simulink model "LED_PWM"  (Simulink 7.5)
settings: Solver=FixedStepDiscrete  SolverMode=SingleTasking  StartTime=0.0  StopTime=10.0  FixedStep=0.001  RelTol=1e-3
libraries: dsPICdrivers x8
settings Model: Creator=oded  LastModifiedBy=oded
settings OptimizationCC: OptimizeModelRefInitCode=on  LifeSpan=1
settings HardwareCC: ProdBitPerInt=16  ProdEndianess=LittleEndian  ProdWordSize=16  ProdHWDeviceType=16-bit Generic
settings RTWCC: SystemTargetFile=dspic.tlc  MakeCommand=make_CreateMPLAB  TemplateMakefile=dspic_pic30_gcc.tmf  PostCodeGenCommand=dsPIC_Compile()  Description=Embedded Target for Microchip dsPIC (real-time)  ProcessScript=dspic_make_rtw_hook
settings CodeAppCC: IgnoreCustomStorageClasses=off
settings STFCustomTargetCC: IncludeMdlTerminateFcn=off  CombineOutputUpdateFcns=on  SuppressErrorStatus=on  ERTCustomFileBanners=on  SupportContinuousTime=off  SupportNonInlinedSFcns=off  SystemTargetFile=dspic.tlc
settings ERTTargetCC: MultiwordLength=2048  ParMdlRefBuildCompliant=off  CompOptLevelCompliant=off  IncludeMdlTerminateFcn=off  SuppressErrorStatus=on  ERTFirstTimeCompliant=off  ModelStepFunctionPrototypeControlCompliant=off  CPPClassGenCompliant=off  InlinedParameterPlacement=NonHierarchical  ERTSrcFileBannerTemplate=dsPIC_code_template.cgt  ERTHdrFileBannerTemplate=dsPIC_code_template.cgt  ERTDataSrcFileTemplate=dsPIC_code_template.cgt  ERTDataHdrFileTemplate=dsPIC_code_template.cgt  ERTCustomFileTemplate=dsPIC_main.tlc  ConvertIfToSwitch=off
settings CustomProperty: DataType=string  Value=C:\PROGRA~1\MATLAB\R2010a\bin\win32\gmake

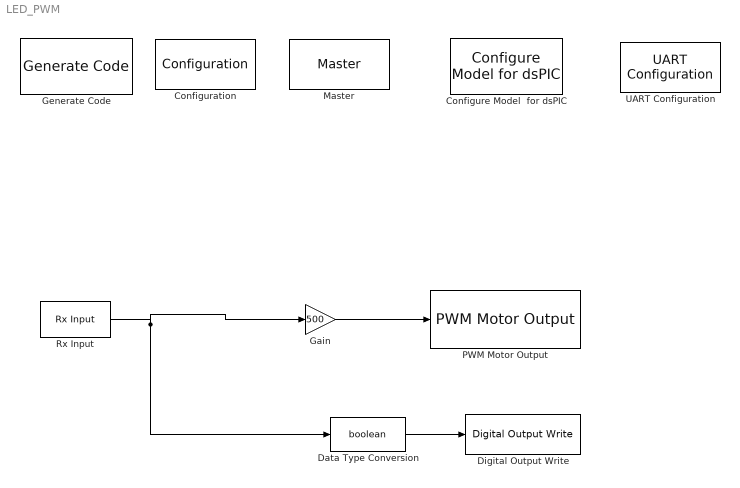
== system LED_PWM ==
  Configuration : dsPICdrivers/Configuration  SystemSampleTime=-1  double64=off
  Configure Model  for dsPIC : dsPICdrivers/Simulink Configuration/Configure Model  for dsPIC
  Data Type Conversion : DataTypeConversion  OutDataTypeMode=boolean  OutDataType=fixdt(1, 16)  OutScaling=2^0  OutDataTypeStr=boolean
  Digital Output Write : dsPICdrivers/Digital I//O/Digital Output Write  Tag=dsPIC_Digital_Output  Priority=5  PORT=B  Pin=[0]  Simultaneous=on  OrderingInOutPopup=None
  Gain : Gain  Gain=500  ParameterDataType=fixdt(1, 16)  ParameterScaling=2^0  OutDataTypeMode=uint16  OutDataType=fixdt(1, 16)  OutScaling=2^0  OutDataTypeStr=uint16
  Generate Code : dsPICdrivers/Simulink Configuration/Generate Code
  Master : dsPICdrivers/Master  Tag=dsPIC_MASTER  Priority=1  TimeStepType=Timer1  picType=30f4011  fcy=5e6  Quartz_33f=5e6  PLLActive_33f=off  fcyDesired_33f=0  tmr1="[1  4999  0]"  tmr1Info="Time Step : 0.001  ;   Error : 0%  PR1=4999"  tmr2345="[0  0  0  0]"  tmr2345cfg=[-1 -1 -1 -1]  IOautoConf=on  typePort="[ 0   0   0   0   0   0   0   0   0   0   0   0   0   0   0   0  10   0   0   0   0   0   0   0   0   0   0   0   0   0   0   0   0   0   0   0   0   0   0   0   0   0   0   0   0   0   0   0   0   0   0   0   0   0   0   0   0   0   0   0   0   0   0   0  11   0   0   0   0   0   0   0   0   0   0   0   0   0   0   0   0   0   0   0   4   5   0   0   0   0   0   0   0   0   0   0   0   0   0   0   0   0   0   0   0   0   0   0   0   0   0   0 ]"  TRIS="[ 65535  65534  65535  65535  65535  65535  65535 ]"  ADPCFG=1  MasterBusyPort=None  MasterOverloadPort=None  FOSC=HS  ClockSwitchMonitor=Both disabled  TempProtection_33f=TEMP_ON  FPBOR=PBOR_OFF  PWRT=PWRT_OFF  MCLR=MCLR_EN  ICD=ICS_PGD1  JTAGEN=JTAGEN_OFF  PowerSave=off  OverrideFcy=off  NewFcy=1e6  PR2345="[65535  65535  65535  65535]"
  PWM Motor Output : dsPICdrivers/Peripheral I//O/PWM Motor Output  Tag=dsPIC_PWM_Motor  Priority=5  PWMref=1  PWM12=1  InputEnableChk=off  InputPeriodeChk=off  Channel=[1 ]  TPeriode=0.02  PrescalerValue=4  PeriodeInteger=25000  MaxName='PWM'  Centered=off  HChannelON=off  Info="Nbr Bits : 15.6096  ||  PWM = 50000  ||  Prescaler = 4"  Delay=0  IntPriority=5  nbrPwmChannelPIC=3  Status=OK  DeadTimePrescaleA=0  DeadTimePrescaleB=0  DeadTimeInfo=Dead Time A = 0  DTPWM1a=Prescaler A  DTPWM1i=Prescaler A  DTPWM2a=Prescaler A  DTPWM2i=Prescaler A  DTPWM3a=Prescaler A  DTPWM3i=Prescaler A  DTPWM4a=Prescaler A  DTPWM4i=Prescaler A  DTCON1=0  DTCON2=0
  Rx Input : dsPICdrivers/Serial PORT/Rx Input  Tag=dsPIC_RX  Priority=5  UART=2  SampleTime=-1  BlockingFctChk=on  OutputDefault=0  IsPresentFlagChk=off  OrderingInOutPopup=None
  UART Configuration : dsPICdrivers/Serial PORT/UART Configuration  Tag=dsPIC_config_UART  Priority=2  UART=2  proposed_BAUD=9600  BAUD=9600  ALT_TX_RX=off  InterruptTxWhen=Do not use interrupt  TXInterruptPri=7  TxBufferSize=32  TXEN=on  InterruptRxWhen=Do not use interrupt  RXInterruptPri=2  RxBufferSize=32  DoNotImplementRxInterrupt=on  DoNotImplementTxInterrupt=on  UxBRG=32  Info="UxBRG = 32   ||  Real Baud : 9470   ||  % error : -1.3573  ||  max 0.94697 Bytes / Step"  RealBaud=0  ERROR=-1.3573  BYTES_STEP=0.94697
  wires:
  Data Type Conversion/1 -> Digital Output Write/1
  Gain/1 -> PWM Motor Output/1
  Rx Input/1 -> Gain/1, Data Type Conversion/1
